simulink model "AmplitudeModulationAndDemodulation1"  (R2025a)
settings: Solver=VariableStepAuto  StartTime=0.0  StopTime=10.0  RelTol=1e-3
libraries: dspfdesign x1
settings Model: Creator=Aman  LastModifiedBy=Aman

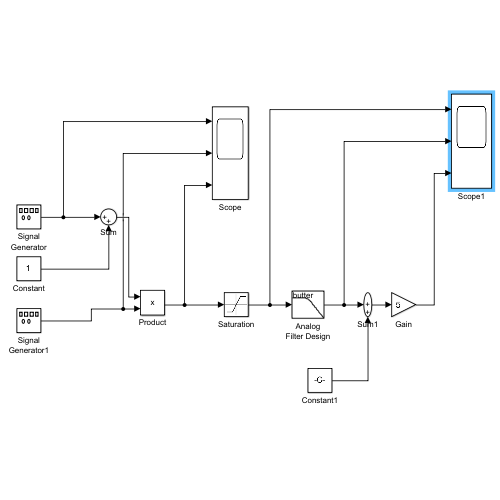
[thumbnail: Simulink's stored preview of the top-level diagram]
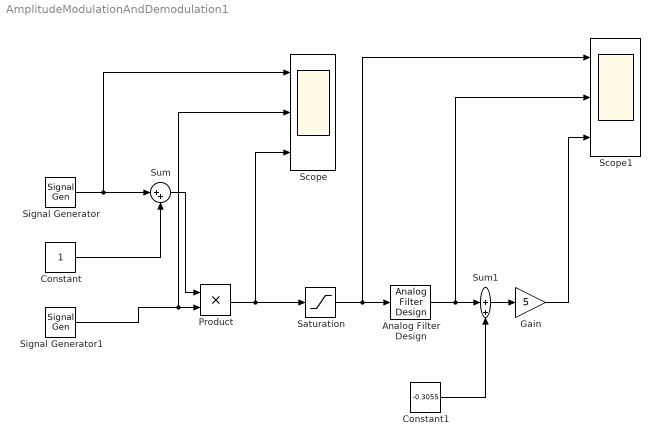
== system AmplitudeModulationAndDemodulation1 ==
  Analog Filter Design : dspfdesign/Analog Filter Design  method=Butterworth  filttype=Lowpass  N=3  Wlo=100  Whi=80  Rp=2  Rs=40
  Constant : Constant
  Constant1 : Constant  Value=-0.3055  SampleTime=0.001
  Gain : Gain  Gain=5
  Product : Product
  Saturation : Saturate  UpperLimit=3  LowerLimit=0
  Scope : Scope  NumInputPorts=3
      settings: ActiveDisplayYMinimum=-7.9285082022906579  ActiveDisplayYMaximum=1.394295407062669
  Scope1 : Scope  NumInputPorts=3
      settings: ActiveDisplayYMinimum=-7.77219209480156  ActiveDisplayYMaximum=1.7292240257911837
  Signal Generator : SignalGenerator  Amplitude=0.5  Frequency=5
  Signal Generator1 : SignalGenerator  Frequency=100
  Sum : Sum  Inputs=|++
  Sum1 : Sum  Inputs=|++
  wires:
  Signal Generator/1 -> Scope/1, Sum/1
  Constant/1 -> Sum/2
  Signal Generator1/1 -> Scope/2, Product/2
  Sum/1 -> Product/1
  Product/1 -> Scope/3, Saturation/1
  Analog Filter Design/1 -> Scope1/2, Sum1/1
  Sum1/1 -> Gain/1
  Saturation/1 -> Scope1/1, Analog Filter Design/1
  Gain/1 -> Scope1/3
  Constant1/1 -> Sum1/2
